simulink model "plant_vertical"  (R2026b)
settings: Solver=VariableStepAuto
undefined symbols (not defined in the file): p
settings Model: Creator=lorenzomonti  LastModifiedBy=lorenzomonti

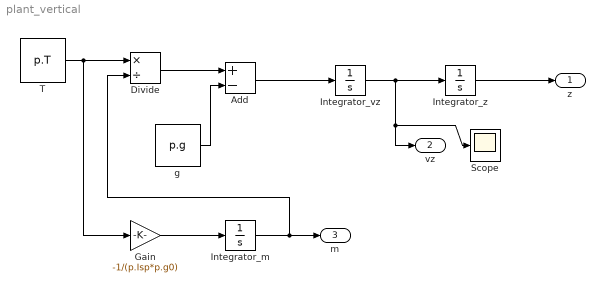
== system plant_vertical ==
  Add : Sum  Inputs=+-
  Divide : Product  Inputs=*/
  Gain : Gain  Gain=-1/(p.Isp*p.g0)
  Integrator_m : Integrator  InitialCondition=p.m0
  Integrator_vz : Integrator  InitialCondition=p.vz0
  Integrator_z : Integrator  InitialCondition=p.z0
  Scope : Scope
      settings: ActiveDisplayYMinimum=-108.3480557337425  ActiveDisplayYMaximum=-24.867498396317547
  T : Constant  Value=p.T
  g : Constant  Value=p.g
  z : Outport
  vz : Outport  Port=2
  m : Outport  Port=3
  wires:
  T/1 -> Gain/1, Divide/1
  Divide/1 -> Add/1
  g/1 -> Add/2
  Add/1 -> Integrator_vz/1
  Integrator_vz/1 -> Scope/1, vz/1, Integrator_z/1
  Integrator_z/1 -> z/1
  Integrator_m/1 -> Divide/2, m/1
  Gain/1 -> Integrator_m/1
